simulink library "simple_wing_lib"  (R2018b)
settings: Solver=VariableStepAuto  StartTime=0.0  StopTime=10.0  RelTol=1e-3
values from neighbouring files (symbols this model uses):
  wing = simpleWingSetYawRateRed( wing )    [simpleWingLoadParams.m]
undefined symbols (not defined in the file or in its folder): wingStruct
libraries: axes_transformation_lib x1, $bdroot x1
settings Model: Creator=Ybeyer  LastModifiedBy=yannic
settings SFSimCC: SimUseLocalCustomCode=off
settings RTWCC: RTWUseLocalCustomCode=off
settings CodeAppCC: StateflowObjectComments=on

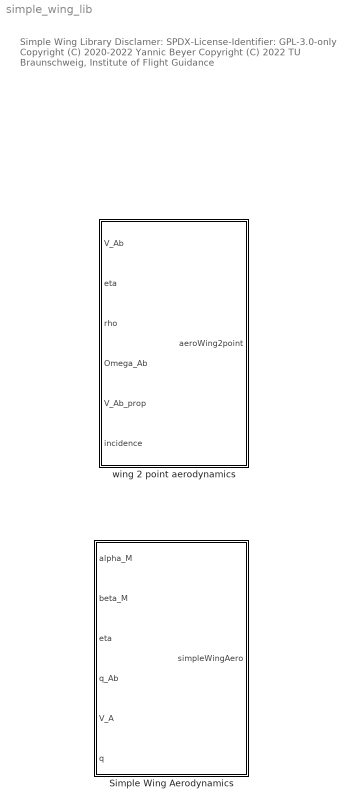
== system simple_wing_lib ==
  note: Simple Wing Library
      |
      | Disclamer:
      | SPDX-License-Identifier: GPL-3.0-only
      |
      | Copyright (C) 2020-2022 Yannic Beyer
      | Copyright (C) 2022 TU Braunschweig, Institute of Flight Guidance
  Simple Wing Aerodynamics : Subsystem  mask{wingStruct=wingStruct}
      mask prompts: wingStruct "simple wing struct"
      mask init:
      | struct2slbus( wingStruct, 'simpleWing' );
      | 
      | % bus objects can not be initialized block workspace and must be moved
      | % to the base workspace
      | % if ~evalin('base','exist(''simpleWingBus'')')
      | %     assignin('base','simpleWingBus',simpleWingBus);
      | % end
      | % clear simpleWingBus;
      mask DialogControl DescGroupVar Prompt: Simple Wing Aerodynamics
      mask DialogControl DescTextVar Prompt: To init a simple wing struct see loadSimpleWingParams.
  wing 2 point aerodynamics : Subsystem  mask{wingStruct=wing, xyz_wing_c=zeros(3,1), xyz_cg_c=zeros(3,1)}
      mask prompts: wingStruct "wing struct containing all relevant parameters"; xyz_wing_c "wing position (c/4 root) in c frame"; xyz_cg_c "CoG position in c frame"
      mask DialogControl DescGroupVar Prompt: wing 2 point aerodynamics
      mask DialogControl DescTextVar Prompt: To init a simple wing struct see loadSimpleWingParams.

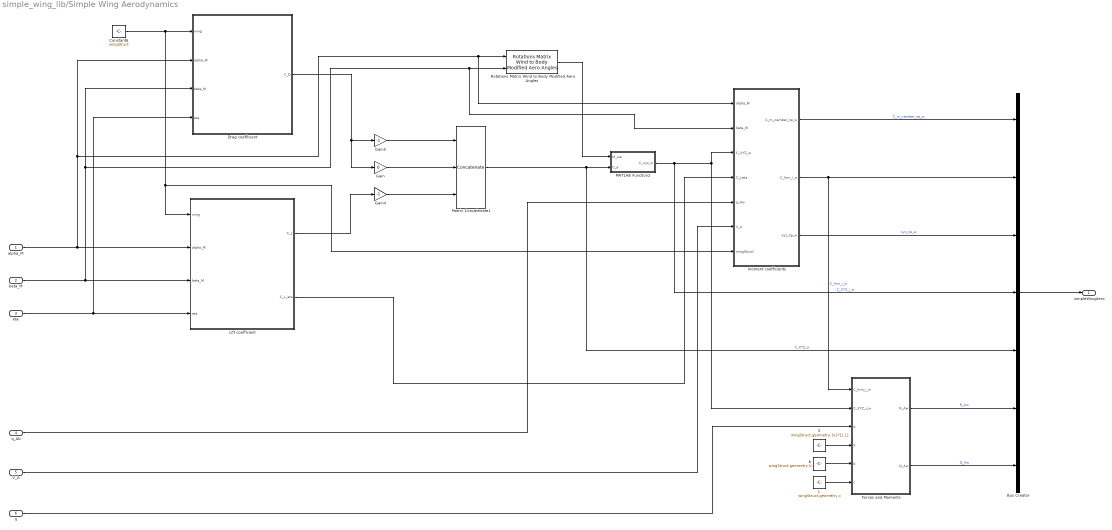
== system simple_wing_lib/Simple Wing Aerodynamics ==
  alpha_M : Inport
  beta_M : Inport  Port=2
  eta : Inport  Port=3
  q_Ab : Inport  Port=4
  V_A : Inport  Port=5
  q : Inport  Port=6
  Bus Creator : BusCreator  Inputs=7
  Constant6 : Constant  Value=wingStruct  OutDataTypeStr=Bus: simpleWingBus
  Drag coefficient : MATLAB Function  TreatAsAtomicUnit=on
  Forces and Moments : MATLAB Function  TreatAsAtomicUnit=on
  Gain : Gain  Gain=0
  Gain4 : Gain  Gain=-1
  Gain5 : Gain  Gain=-1
  Lift coefficient : MATLAB Function  TreatAsAtomicUnit=on
  MATLAB Function2 : MATLAB Function  TreatAsAtomicUnit=on
  Matrix Concatenate1 : Concatenate  NumInputs=3  Mode=Multidimensional array
  Rotations Matrix Wind to Body Modified Aero Angles : axes_transformation_lib/Rotations Matrix Wind to Body Modified Aero Angles  SystemSampleTime=-1
      settings: SourceProductName=LADAC
  S : Constant  Value=wingStruct.geometry.S/2*[1,1]  VectorParams1D=off
  b : Constant  Value=wingStruct.geometry.b
  c : Constant  Value=wingStruct.geometry.c
  moment coefficients : Subsystem
  simpleWingAero : Outport
  wires:
  Gain4/1 -> Matrix Concatenate1/3
  Gain5/1 -> Matrix Concatenate1/1
  Gain/1 -> Matrix Concatenate1/2
  beta_M/1 -> moment coefficients/2(beta_M), Rotations Matrix Wind to Body Modified Aero Angles/2, Drag coefficient/3(beta_M), Lift coefficient/3(beta_M)
  eta/1 -> Drag coefficient/4(eta), Lift coefficient/4(eta)
  Constant6/1 -> Lift coefficient/1(wing), moment coefficients/7(wingStruct), Drag coefficient/1(wing)
  Lift coefficient/1(C_L) -> Gain4/1
  Drag coefficient/1(C_D) -> Gain/1, Gain5/1
  alpha_M/1 -> moment coefficients/1(alpha_M), Rotations Matrix Wind to Body Modified Aero Angles/1, Drag coefficient/2(alpha_M), Lift coefficient/2(alpha_M)
  Matrix Concatenate1/1 -> Bus Creator/5, MATLAB Function2/2(C_a)  "C_XYZ_a"
  Rotations Matrix Wind to Body Modified Aero Angles/1 -> MATLAB Function2/1(M_wa)
  moment coefficients/2(C_lmn_i_w) -> Forces and Moments/1(C_lmn_i_w), Bus Creator/2  "C_lmn_i_w"
  MATLAB Function2/1(C_xyz_w) -> Bus Creator/4, Forces and Moments/2(C_XYZ_i_w), moment coefficients/3(C_XYZ_w)  "C_XYZ_i_w"
  moment coefficients/1(C_m_camber_np_w) -> Bus Creator/1  "C_m_camber_np_w"
  Lift coefficient/2(C_L_eta) -> moment coefficients/4(C_Leta)
  moment coefficients/3(xyz_np_w) -> Bus Creator/3  "xyz_np_w"
  q_Ab/1 -> moment coefficients/5(q_Aw)
  V_A/1 -> moment coefficients/6(V_A)
  Bus Creator/1 -> simpleWingAero/1
  q/1 -> Forces and Moments/3(q)
  S/1 -> Forces and Moments/4(S)
  b/1 -> Forces and Moments/5(b)
  c/1 -> Forces and Moments/6(c)
  Forces and Moments/1(R_Aw) -> Bus Creator/6  "R_Aw"
  Forces and Moments/2(Q_Aw) -> Bus Creator/7  "Q_Aw"

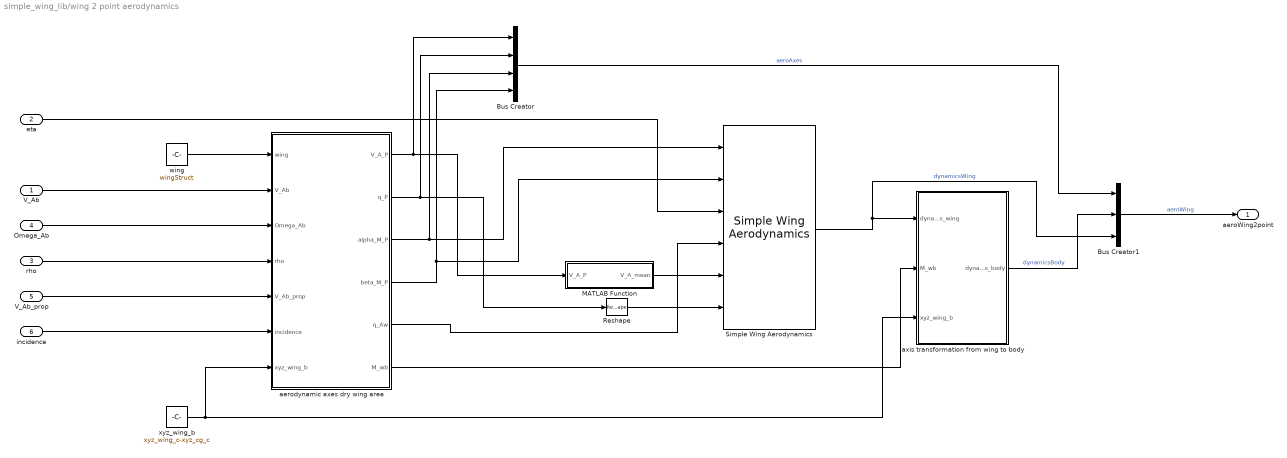
== system simple_wing_lib/wing 2 point aerodynamics ==
  V_Ab : Inport
  eta : Inport  Port=2
  rho : Inport  Port=3
  Omega_Ab : Inport  Port=4
  V_Ab_prop : Inport  Port=5
  incidence : Inport  Port=6
  Bus Creator : BusCreator  Inputs=4
  Bus Creator1 : BusCreator  Inputs=3
  MATLAB Function : MATLAB Function  TreatAsAtomicUnit=on
  Reshape : Reshape  OutputDimensionality=Row vector (2-D)
  Simple Wing Aerodynamics : $bdroot/Simple Wing Aerodynamics  wingStruct=wingStruct
  aerodynamic axes dry wing area : MATLAB Function  TreatAsAtomicUnit=on
  axis transformation from wing to body : Subsystem
  wing : Constant  Value=wingStruct  OutDataTypeStr=Bus: simpleWingBus
  xyz_wing_b : Constant  Value=xyz_wing_c-xyz_cg_c  VectorParams1D=off
  aeroWing2point : Outport
  wires:
  aerodynamic axes dry wing area/4(beta_M_P) -> Bus Creator/4, Simple Wing Aerodynamics/2
  Reshape/1 -> Simple Wing Aerodynamics/6
  aerodynamic axes dry wing area/2(q_P) -> Bus Creator/2, Reshape/1
  V_Ab/1 -> aerodynamic axes dry wing area/2(V_Ab)
  rho/1 -> aerodynamic axes dry wing area/4(rho)
  aerodynamic axes dry wing area/3(alpha_M_P) -> Bus Creator/3, Simple Wing Aerodynamics/1
  aerodynamic axes dry wing area/1(V_A_P) -> Bus Creator/1, MATLAB Function/1(V_A_P)
  Simple Wing Aerodynamics/1 -> Bus Creator1/3, axis transformation from wing to body/1(dynamics_wing)  "dynamicsWing"
  eta/1 -> Simple Wing Aerodynamics/3
  wing/1 -> aerodynamic axes dry wing area/1(wing)
  Omega_Ab/1 -> aerodynamic axes dry wing area/3(Omega_Ab)
  MATLAB Function/1(V_A_mean) -> Simple Wing Aerodynamics/5
  aerodynamic axes dry wing area/5(q_Aw) -> Simple Wing Aerodynamics/4
  Bus Creator1/1 -> aeroWing2point/1  "aeroWing"
  Bus Creator/1 -> Bus Creator1/1  "aeroAxes"
  V_Ab_prop/1 -> aerodynamic axes dry wing area/5(V_Ab_prop)
  incidence/1 -> aerodynamic axes dry wing area/6(incidence)
  axis transformation from wing to body/1(dynamics_body) -> Bus Creator1/2  "dynamicsBody"
  aerodynamic axes dry wing area/6(M_wb) -> axis transformation from wing to body/2(M_wb)
  xyz_wing_b/1 -> axis transformation from wing to body/3(xyz_wing_b), aerodynamic axes dry wing area/7(xyz_wing_b)

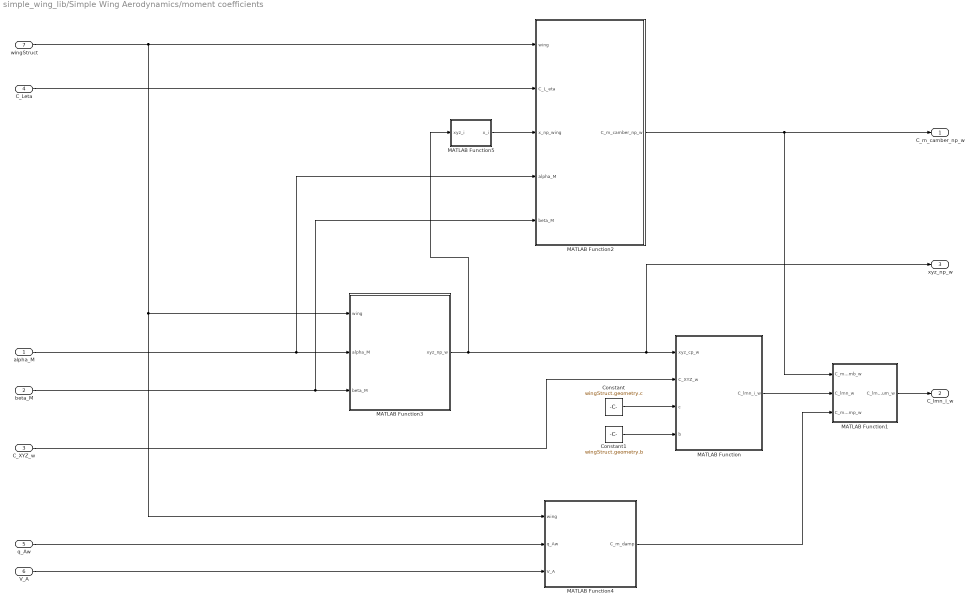
== system simple_wing_lib/Simple Wing Aerodynamics/moment coefficients ==
  alpha_M : Inport
  beta_M : Inport  Port=2
  C_XYZ_w : Inport  Port=3
  C_Leta : Inport  Port=4
  q_Aw : Inport  Port=5
  V_A : Inport  Port=6
  wingStruct : Inport  Port=7
  Constant : Constant  Value=wingStruct.geometry.c
  Constant1 : Constant  Value=wingStruct.geometry.b
  MATLAB Function : MATLAB Function  TreatAsAtomicUnit=on
  MATLAB Function1 : MATLAB Function  TreatAsAtomicUnit=on
  MATLAB Function2 : MATLAB Function  TreatAsAtomicUnit=on
  MATLAB Function3 : MATLAB Function  TreatAsAtomicUnit=on
  MATLAB Function4 : MATLAB Function  TreatAsAtomicUnit=on
  MATLAB Function5 : MATLAB Function  TreatAsAtomicUnit=on
  C_m_camber_np_w : Outport
  C_lmn_i_w : Outport  Port=2
  xyz_np_w : Outport  Port=3
  wires:
  MATLAB Function3/1(xyz_np_w) -> MATLAB Function5/1(xyz_i), xyz_np_w/1, MATLAB Function/1(xyz_cp_w)
  beta_M/1 -> MATLAB Function2/5(beta_M), MATLAB Function3/3(beta_M)
  alpha_M/1 -> MATLAB Function3/2(alpha_M), MATLAB Function2/4(alpha_M)
  C_Leta/1 -> MATLAB Function2/2(C_L_eta)
  MATLAB Function2/1(C_m_camber_np_w) -> MATLAB Function1/1(C_m_camb_w), C_m_camber_np_w/1
  C_XYZ_w/1 -> MATLAB Function/2(C_XYZ_w)
  MATLAB Function/1(C_lmn_i_w) -> MATLAB Function1/2(C_lmn_w)
  Constant/1 -> MATLAB Function/3(c)
  Constant1/1 -> MATLAB Function/4(b)
  MATLAB Function1/1(C_lmn_sum_w) -> C_lmn_i_w/1
  MATLAB Function4/1(C_m_damp) -> MATLAB Function1/3(C_m_damp_w)
  q_Aw/1 -> MATLAB Function4/2(q_Aw)
  V_A/1 -> MATLAB Function4/3(V_A)
  wingStruct/1 -> MATLAB Function4/1(wing), MATLAB Function3/1(wing), MATLAB Function2/1(wing)
  MATLAB Function5/1(x_i) -> MATLAB Function2/3(x_np_wing)

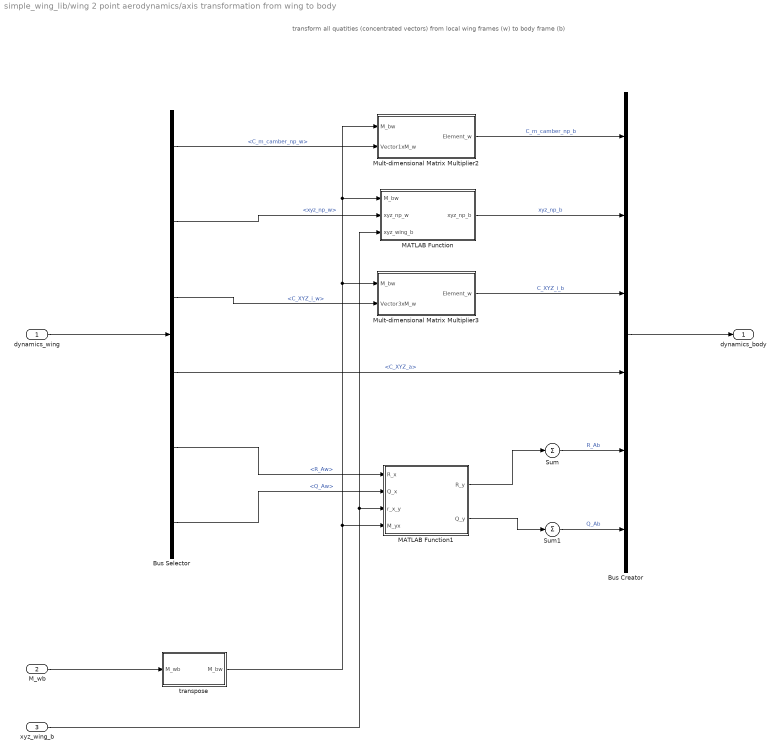
== system simple_wing_lib/wing 2 point aerodynamics/axis transformation from wing to body ==
  note: transform all quatities (concentrated vectors) from local wing frames (w) to body frame (b)
  dynamics_wing : Inport
  M_wb : Inport  Port=2
  xyz_wing_b : Inport  Port=3
  Bus Creator : BusCreator  Inputs=6
  Bus Selector : BusSelector  OutputSignals=C_m_camber_np_w,xyz_np_w,C_XYZ_i_w,C_XYZ_a,R_Aw,Q_Aw
  MATLAB Function : MATLAB Function  TreatAsAtomicUnit=on
  MATLAB Function1 : MATLAB Function  TreatAsAtomicUnit=on
  Mult-dimensional Matrix Multiplier2 : MATLAB Function  TreatAsAtomicUnit=on
  Mult-dimensional Matrix Multiplier3 : MATLAB Function  TreatAsAtomicUnit=on
  Sum : Sum  Inputs=+  CollapseMode=Specified dimension  CollapseDim=2
  Sum1 : Sum  Inputs=+  CollapseMode=Specified dimension  CollapseDim=2
  transpose : MATLAB Function  TreatAsAtomicUnit=on
  dynamics_body : Outport
  wires:
  dynamics_wing/1 -> Bus Selector/1
  M_wb/1 -> transpose/1(M_wb)
  Bus Selector/1 -> Mult-dimensional Matrix Multiplier2/2(Vector1xM_w)  "<C_m_camber_np_w>"
  Bus Selector/3 -> Mult-dimensional Matrix Multiplier3/2(Vector3xM_w)  "<C_XYZ_i_w>"
  Bus Selector/5 -> MATLAB Function1/1(R_x)  "<R_Aw>"
  Bus Selector/6 -> MATLAB Function1/2(Q_x)  "<Q_Aw>"
  MATLAB Function/1(xyz_np_b) -> Bus Creator/2  "xyz_np_b"
  Mult-dimensional Matrix Multiplier3/1(Element_w) -> Bus Creator/3  "C_XYZ_i_b"
  Bus Selector/4 -> Bus Creator/4  "<C_XYZ_a>"
  MATLAB Function1/1(R_y) -> Sum/1
  MATLAB Function1/2(Q_y) -> Sum1/1
  Bus Creator/1 -> dynamics_body/1
  transpose/1(M_bw) -> Mult-dimensional Matrix Multiplier3/1(M_bw), Mult-dimensional Matrix Multiplier2/1(M_bw), MATLAB Function/1(M_bw), MATLAB Function1/4(M_yx)
  Bus Selector/2 -> MATLAB Function/2(xyz_np_w)  "<xyz_np_w>"
  Mult-dimensional Matrix Multiplier2/1(Element_w) -> Bus Creator/1  "C_m_camber_np_b"
  Sum/1 -> Bus Creator/5  "R_Ab"
  Sum1/1 -> Bus Creator/6  "Q_Ab"
  xyz_wing_b/1 -> MATLAB Function/3(xyz_wing_b), MATLAB Function1/3(r_x_y)

== matlab function simple_wing_lib/Simple Wing Aerodynamics/moment coefficients/MATLAB Function5 ==
  data: xyz_i input; x_i output
function x_i = fcn(xyz_i)

x_i = xyz_i(1,:);

== matlab function simple_wing_lib/wing 2 point aerodynamics/MATLAB Function ==
  data: V_A_P input; V_A_mean output
function V_A_mean  = fcn(V_A_P) %#codegen
    V_A_mean = mean( V_A_P);
end

== matlab function simple_wing_lib/wing 2 point aerodynamics/aerodynamic axes dry wing area ==
  data: wing input; V_Ab input; V_A_P output; q_P output; alpha_M_P output; beta_M_P output; Omega_Ab input; rho input; V_Ab_prop input; incidence input; q_Aw output; M_wb output; xyz_wing_b input
function [ V_A_P, q_P, alpha_M_P, beta_M_P, q_Aw, M_wb ] = ...
    simpleWingGetInflow( wing, V_Ab, Omega_Ab, rho, V_Ab_prop, ...
    incidence,  xyz_wing_b )
[ V_A_P, q_P, alpha_M_P, beta_M_P, q_Aw, M_wb ] = ...
    simpleWingGetInflow( wing, V_Ab, Omega_Ab, rho, V_Ab_prop, ...
    incidence, xyz_wing_b );
end

== matlab function simple_wing_lib/wing 2 point aerodynamics/axis transformation from wing to body/MATLAB Function ==
  data: M_bw input; xyz_np_b output; xyz_np_w input; xyz_wing_b input
function xyz_np_b = fcn(M_bw,xyz_np_w,xyz_wing_b)
xyz_np_b = zeros(size(xyz_np_w));
for i = 1:size(xyz_np_w,2)
    xyz_np_b(:,i) = xyz_np_w(:,i) + M_bw(:,:,i)*xyz_wing_b;
end

== matlab function simple_wing_lib/wing 2 point aerodynamics/axis transformation from wing to body/MATLAB Function1 ==
  data: R_x input; R_y output; Q_x input; r_x_y input; M_yx input; Q_y output
function [ R_y, Q_y ] = fcn( R_x, Q_x, r_x_y, M_yx )%#codegen
R_y = zeros(size(R_x));
Q_y = zeros(size(R_x));
for i = 1:size(R_x,2)
    [ R_y(:,i), Q_y(:,i) ] = forceMomentTransform( R_x(:,i), Q_x(:,i), ...
        r_x_y, M_yx(:,:,i) );
end

== matlab function simple_wing_lib/wing 2 point aerodynamics/axis transformation from wing to body/Mult-dimensional Matrix Multiplier2 ==
  data: M_bw input; Element_w output; Vector1xM_w input
function Element_w = fcn(M_bw,Vector1xM_w)
len = length(Vector1xM_w(1,:));
Element_w = zeros(3,len);
for i = 1:len
    Element_w(:,i) = M_bw(:,2,i) * Vector1xM_w(:,i);    
end
end

== matlab function simple_wing_lib/Simple Wing Aerodynamics/Drag coefficient ==
  data: wing input; C_D output; alpha_M input; beta_M input; eta input
function C_D = fcn( wing, alpha_M, beta_M, eta ) %#codegen

C_D = simpleWingGetCd( wing, alpha_M, beta_M, eta );

end

== matlab function simple_wing_lib/wing 2 point aerodynamics/axis transformation from wing to body/Mult-dimensional Matrix Multiplier3 ==
  data: M_bw input; Element_w output; Vector3xM_w input
function Element_w = fcn(M_bw,Vector3xM_w)
len = length(Vector3xM_w(1,:));
Element_w = zeros(3,len);
for i = 1:len
    Element_w(:,i) = M_bw(:,:,i) * Vector3xM_w(:,i);    
end
end

== matlab function simple_wing_lib/Simple Wing Aerodynamics/Forces and Moments ==
  data: C_lmn_i_w input; R_Aw output; C_XYZ_i_w input; q input; S input; b input; c input; Q_Aw output
function [ R_Aw, Q_Aw ] = fcn( C_lmn_i_w, C_XYZ_i_w, ...
    q, S, b, c ) %#codegen
    R_Aw = zeros( size( C_XYZ_i_w ) );
    Q_Aw = zeros( size( C_XYZ_i_w ) );
    for i = 1:size(C_XYZ_i_w,2)
        [ R_Aw(:,i), Q_Aw(:,i) ] = coeffs2ForcesMoments( ...
            C_lmn_i_w(:,i), C_XYZ_i_w(:,i), q(:,i), S(:,i), b, c );
    end
end

== matlab function simple_wing_lib/wing 2 point aerodynamics/axis transformation from wing to body/transpose ==
  data: M_wb input; M_bw output
function M_bw = fcn(M_wb) %#codegen
M_bw = permute( M_wb, [2,1,3] );
end

== matlab function simple_wing_lib/Simple Wing Aerodynamics/Lift coefficient ==
  data: wing input; C_L output; alpha_M input; beta_M input; eta input; C_L_eta output
function [ C_L, C_L_eta ] = simpleWingGetCl( wing, alpha_M, beta_M, eta )  %#codegen

[ C_L, C_L_eta ] = simpleWingGetCl( wing, alpha_M, beta_M, eta );

end

== matlab function simple_wing_lib/Simple Wing Aerodynamics/MATLAB Function2 ==
  data: M_wa input; C_xyz_w output; C_a input
function C_xyz_w = fcn(M_wa,C_a)

len = length(C_a(1,:));
C_xyz_w = zeros(3,len);

for i = 1:len
    C_xyz_w(:,i) = M_wa(:,:,i) * C_a(:,i);    
end

end

== matlab function simple_wing_lib/Simple Wing Aerodynamics/moment coefficients/MATLAB Function ==
  data: xyz_cp_w input; C_XYZ_w input; C_lmn_i_w output; c input; b input
function C_lmn_i_w = forceCoeffs2MomentCoeffs( xyz_cp_w, C_XYZ_w, c, b ) %#codegen
[ C_lmn_i_w ] = forceCoeffs2MomentCoeffs( xyz_cp_w, C_XYZ_w, c, b );
end

== matlab function simple_wing_lib/Simple Wing Aerodynamics/moment coefficients/MATLAB Function1 ==
  data: C_m_camb_w input; C_lmn_sum_w output; C_lmn_w input; C_m_damp_w input
function C_lmn_sum_w = fcn(C_m_camb_w,C_lmn_w, C_m_damp_w) %#codegen
% sum of all moment coefficients in wing (w) frame

C_lmn_sum_w = C_lmn_w;
C_lmn_sum_w(2,:) = C_lmn_w(2,:) + C_m_camb_w + C_m_damp_w;

end

== matlab function simple_wing_lib/Simple Wing Aerodynamics/moment coefficients/MATLAB Function2 ==
  data: wing input; C_m_camber_np_w output; C_L_eta input; x_np_wing input; alpha_M input; beta_M input
function C_m_camber_np_w = simpleWingGetCmCamber( wing, C_L_eta, x_np_wing, alpha_M, beta_M ) %#codegen
[ C_m_camber_np_w ] = simpleWingGetCmCamber( wing, C_L_eta, x_np_wing, alpha_M, beta_M );
end

== matlab function simple_wing_lib/Simple Wing Aerodynamics/moment coefficients/MATLAB Function3 ==
  data: wing input; xyz_np_w output; alpha_M input; beta_M input
function xyz_np_w = simpleWingGetNeutralPoint( wing, alpha_M, beta_M )
[ xyz_np_w ] = simpleWingGetNeutralPoint( wing, alpha_M, beta_M );
end

== matlab function simple_wing_lib/Simple Wing Aerodynamics/moment coefficients/MATLAB Function4 ==
  data: wing input; C_m_damp output; q_Aw input; V_A input
function C_m_damp = simpleWingGetPitchDamping( wing, q_Aw, V_A ) %#codegen
    C_m_damp = simpleWingGetPitchDamping( wing, q_Aw, V_A );
end
